simulink model "FlexBoard_Blinking_Led"  (Simulink 6.4)
settings: Solver=FixedStepDiscrete  StartTime=0.0  StopTime=10.0  FixedStep=0.002  RelTol=1e-3
libraries: dsPICdrivers x8, simulink x4
settings Model: Creator=Lubin  LastModifiedBy=Lubin
settings DataIOCC: SaveOutput=off  SaveTime=off
settings OptimizationCC: InlineParams=on  InlineInvariantSignals=on  EnforceIntegerDowncast=off  StateBitsets=on  DataBitsets=on  UseTempVars=on  ZeroExternalMemoryAtStartup=off  ZeroInternalMemoryAtStartup=off  InitFltsAndDblsToZero=off  NoFixptDivByZeroProtection=on  EfficientFloat2IntCast=on  OptimizeModelRefInitCode=on  LifeSpan=1
settings DebuggingCC: MultiTaskDSMMsg=error  MultiTaskCondExecSysMsg=error
settings HardwareCC: ProdBitPerInt=16  ProdEndianess=LittleEndian  ProdWordSize=16  ProdHWDeviceType=16-bit Generic  TargetHWDeviceType=32-bit Generic
settings RTWCC: SystemTargetFile=dspic.tlc  TemplateMakefile=dspic_pic30_gcc.tmf  PostCodeGenCommand=dsPIC_Compile()  Description=Embedded Target for Microchip dsPIC (real-time)  GenerateReport=on  RTWVerbose=off  ProcessScript=dspic_make_rtw_hook  IncludeHyperlinkInReport=on  LaunchReport=on
settings CodeAppCC: ForceParamTrailComments=on  IgnoreCustomStorageClasses=off  SimulinkDataObjDesc=on  CustomSymbolStrGlobalVar=rt$N$M  CustomSymbolStrType=$N$M  CustomSymbolStrFcn=$N$M$F  CustomSymbolStrMacro=$N$M  InsertBlockDesc=on
settings STFCustomTargetCC: TargetFcnLib=ansi_tfl_tmw.mat  GenFloatMathFcnCalls=ANSI_C  ModelReferenceCompliant=off  IncludeMdlTerminateFcn=off  CombineOutputUpdateFcns=on  SuppressErrorStatus=on  ERTCustomFileBanners=on  SupportContinuousTime=off  SupportNonInlinedSFcns=off  SystemTargetFile=dspic.tlc
settings ERTTargetCC: TargetFcnLib=ansi_tfl_tmw.mat  GenFloatMathFcnCalls=ANSI_C  ModelReferenceCompliant=off  CompOptLevelCompliant=off  IncludeMdlTerminateFcn=off  SuppressErrorStatus=on  ModelStepFunctionPrototypeControlCompliant=off  InlinedParameterPlacement=NonHierarchical  ERTSrcFileBannerTemplate=dsPIC_code_template.cgt  ERTHdrFileBannerTemplate=dsPIC_code_template.cgt  ERTDataSrcFileTemplate=dsPIC_code_template.cgt  ERTDataHdrFileTemplate=dsPIC_code_template.cgt  ERTCustomFileTemplate=dsPIC_main.tlc
settings CustomProperty: DataType=string  Value=C:\PROGRA~1\MATLAB\R2008a\bin\win32\gmake

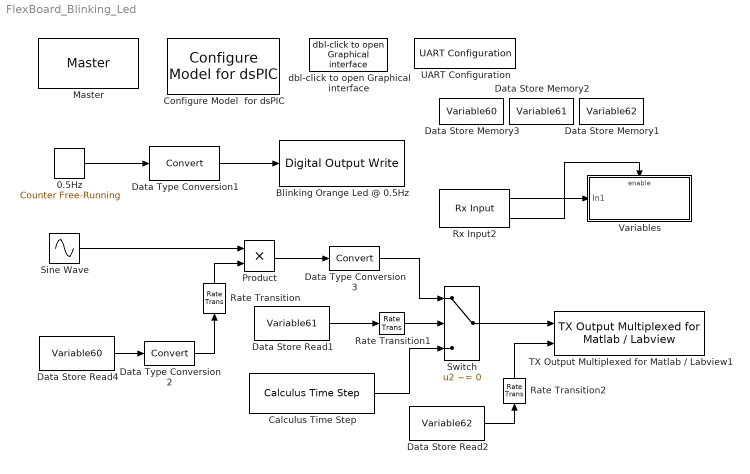
== system FlexBoard_Blinking_Led ==
  0.5Hz : simulink/Sources/Counter Free-Running  SystemSampleTime=-1  NumBits=1  tsamp=.25
  Blinking Orange Led @ 0.5Hz : dsPICdrivers/Digital I//O/Digital Output Write  Tag=dsPIC_Digital_Output  Priority=5  PORT=B  Simultaneous=off  OrderingInOutPopup=None
  Calculus Time Step : dsPICdrivers/OTHERS/Calculus Time Step  Tag=dsPIC_CalculusTimeStep  SampleTime=-1  PR1chk=off
  Configure Model  for dsPIC : dsPICdrivers/Simulink Configuration/Configure Model  for dsPIC
  Data Store Memory1 : DataStoreMemory  DataStoreName=Variable62  ReadBeforeWriteMsg=warning  WriteAfterWriteMsg=warning  WriteAfterReadMsg=warning  DataType=uint8  OutDataType=sfix(16)  OutScaling=2^0
  Data Store Memory2 : DataStoreMemory  DataStoreName=Variable61  ReadBeforeWriteMsg=warning  WriteAfterWriteMsg=warning  WriteAfterReadMsg=warning  InitialValue=1  DataType=uint8  OutDataType=sfix(16)  OutScaling=2^0
  Data Store Memory3 : DataStoreMemory  DataStoreName=Variable60  ReadBeforeWriteMsg=warning  WriteAfterWriteMsg=warning  WriteAfterReadMsg=warning  InitialValue=255  DataType=uint8  OutDataType=sfix(16)  OutScaling=2^0
  Data Store Read1 : DataStoreRead  DataStoreName=Variable61  SampleTime=.01
  Data Store Read2 : DataStoreRead  DataStoreName=Variable62  SampleTime=.01
  Data Store Read4 : DataStoreRead  DataStoreName=Variable60  SampleTime=.01
  Data Type Conversion1 : DataTypeConversion  OutDataTypeMode=boolean  OutDataType=sfix(16)  OutScaling=2^0
  Data Type Conversion2 : DataTypeConversion  OutDataTypeMode=double  OutDataType=sfix(16)  OutScaling=2^0
  Data Type Conversion3 : DataTypeConversion  OutDataTypeMode=int16  OutDataType=sfix(16)  OutScaling=2^0
  Master : dsPICdrivers/Master  Tag=dsPIC_MASTER  Priority=1  TimeStepType=Timer1  picType=33fJ256MC710  fcy=9200000  Quartz_33f=4e6  PLLActive_33f=on  fcyDesired_33f=9.2e6  tmr1="[1  18399  0]"  tmr1Info="Time Step : 0.002  ;   Error : 0%  PR1=18399"  tmr2345="[0  0  0  0  0  0  0  0]"  tmr2345cfg=[-1 -1 -1 -1 -1 -1 -1 -1]  IOautoConf=on  typePort="[ 0   0   0   0   0   0   0   0   0   0   0   0   0   0   0   0   0   0   0   0   0   0   0   0   0   0   0   0   0   0  10   0   0   0   0   0   0   0   0   0   0   0   0   0   0   0   0   0   0   0   0   0   0   0   0   0   0   0   0   0   0   0   0   0   0   0   0   0   0   0   0   0   0   0   0   0   0   0   0   0   0   0   4   5   0   0   0   0   0   0   0   0   0   0   0   0   0   0   0   0   0   0   0   0   0   0   0   0   0   0   0   0 ]"  TRIS="[ 65535  49151  65535  65535  65535  65535  65535 ]"  ADPCFG=16384  MasterBusyPort=None  MasterOverloadPort=None  FOSC=Quartz (XT - HS)  TempProtection_33f=TEMP_ON  FPBOR=<empty>  PWRT=32ms  MCLR=<empty>  PowerSave=off
  Product : Product  OutDataType=sfix(16)  OutScaling=2^0  RndMeth=Zero
  Rate Transition : RateTransition  Orientation=up  Integrity=off  Deterministic=off
  Rate Transition1 : RateTransition  Integrity=off  Deterministic=off
  Rate Transition2 : RateTransition  Orientation=up  Integrity=off  Deterministic=off
  Rx Input2 : dsPICdrivers/Serial PORT/Rx Input  Tag=dsPIC_RX  Priority=5  UART=1  SampleTime=.01  BlockingFctChk=off  OutputDefault=0  IsPresentFlagChk=on
  Sine Wave : Sin  SineType=Sample based  Frequency=6  Samples=500  SampleTime=.002
  Switch : Switch  Criteria=u2 ~= 0
  TX Output Multiplexed for Matlab / Labview1 : dsPICdrivers/Serial PORT/TX Output Multiplexed for Matlab // Labview  Tag=dsPIC_TX_Multiplexed  Priority=5  UART=1  CleverSpreadingChk=on  CleverSpreading=1  CHANNEL=[0 1 ]  CHANNELBLOCKED=[]  CHANNELBLOCKED_BITEWISE=0  Status=OK
  UART Configuration : dsPICdrivers/Serial PORT/UART Configuration  Tag=dsPIC_config_UART  Priority=2  UART=1  proposed_BAUD=115200  ALT_TX_RX=off  InterruptTxWhen=When Transmit Buffer is empty  TXInterruptPri=1  TxBufferSize=32  TXEN=on  InterruptRxWhen=When Receive Buffer is 3/4 full (contain 3 characters)  RXInterruptPri=5  RxBufferSize=32  BAUD=115200  UxBRG=4  Info="UxBRG = 4   ||  Real Baud : 115000   ||  % error : -0.17361  ||  max 23 Bytes / Step"  RealBaud=0
  Variables : Subsystem  TreatAsAtomicUnit=on
  dbl-click to open Graphical interface : dsPICdrivers/Serial PORT/dbl-click to open Graphical interface  SystemSampleTime=-1  Nothing=0
  wires:
  0.5Hz/1 -> Data Type Conversion1/1
  Data Type Conversion1/1 -> Blinking Orange Led @ 0.5Hz/1
  Rx Input2/1 -> Variables/1(In1)
  Rx Input2/2 -> Variables/Enable
  Sine Wave/1 -> Product/1
  Data Store Read4/1 -> Data Type Conversion2/1
  Data Type Conversion2/1 -> Rate Transition/1
  Product/1 -> Data Type Conversion3/1
  Data Store Read1/1 -> Rate Transition1/1
  Switch/1 -> TX Output Multiplexed for Matlab / Labview1/1
  Data Type Conversion3/1 -> Switch/1
  Calculus Time Step/1 -> Switch/3
  Data Store Read2/1 -> Rate Transition2/1
  Rate Transition/1 -> Product/2
  Rate Transition1/1 -> Switch/2
  Rate Transition2/1 -> TX Output Multiplexed for Matlab / Labview1/2

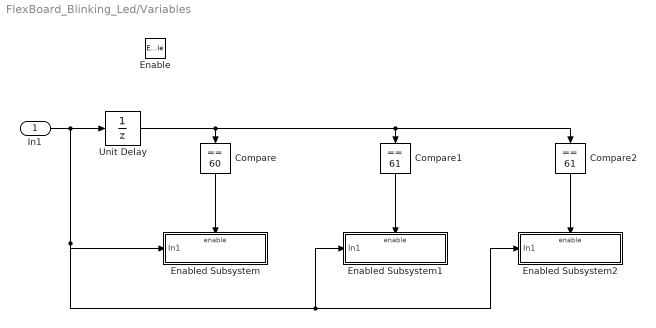
== system FlexBoard_Blinking_Led/Variables ==
  In1 : Inport  OutDataType=sfix(16)  OutScaling=2^0
  Enable : EnablePort
  Compare : simulink/Logic and Bit Operations/Compare To Constant  Orientation=down  SystemSampleTime=-1  relop===  const=60  LogicOutDataTypeMode=boolean  ZeroCross=off
  Compare1 : simulink/Logic and Bit Operations/Compare To Constant  Orientation=down  SystemSampleTime=-1  relop===  const=61  LogicOutDataTypeMode=boolean  ZeroCross=off
  Compare2 : simulink/Logic and Bit Operations/Compare To Constant  Orientation=down  SystemSampleTime=-1  relop===  const=61  LogicOutDataTypeMode=boolean  ZeroCross=off
  Enabled Subsystem : Subsystem  TreatAsAtomicUnit=on
  Enabled Subsystem1 : Subsystem  TreatAsAtomicUnit=on
  Enabled Subsystem2 : Subsystem  TreatAsAtomicUnit=on
  Unit Delay : UnitDelay  SampleTime=-1
  wires:
  Compare2/1 -> Enabled Subsystem2/Enable
  In1/1 -> Unit Delay/1, Enabled Subsystem2/1(In1), Enabled Subsystem1/1(In1), Enabled Subsystem/1(In1)
  Unit Delay/1 -> Compare2/1, Compare1/1, Compare/1
  Compare/1 -> Enabled Subsystem/Enable
  Compare1/1 -> Enabled Subsystem1/Enable

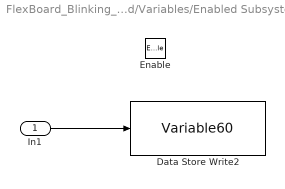
== system FlexBoard_Blinking_Led/Variables/Enabled Subsystem ==
  In1 : Inport  OutDataType=sfix(16)  OutScaling=2^0
  Enable : EnablePort
  Data Store Write2 : DataStoreWrite  DataStoreName=Variable60  SampleTime=-1
  wires:
  In1/1 -> Data Store Write2/1

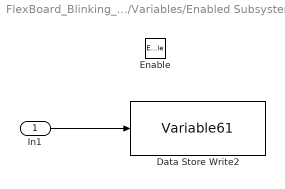
== system FlexBoard_Blinking_Led/Variables/Enabled Subsystem1 ==
  In1 : Inport  OutDataType=sfix(16)  OutScaling=2^0
  Enable : EnablePort
  Data Store Write2 : DataStoreWrite  DataStoreName=Variable61  SampleTime=-1
  wires:
  In1/1 -> Data Store Write2/1

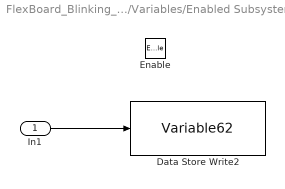
== system FlexBoard_Blinking_Led/Variables/Enabled Subsystem2 ==
  In1 : Inport  OutDataType=sfix(16)  OutScaling=2^0
  Enable : EnablePort
  Data Store Write2 : DataStoreWrite  DataStoreName=Variable62  SampleTime=-1
  wires:
  In1/1 -> Data Store Write2/1
